simulink model "ecu_mode"  (R2026a)
settings: Solver=FixedStepDiscrete  StopTime=10  FixedStep=0.001  SampleTimeConstraint=STIndependent
Description:
  | Engine state machine. Source of truth for firmware/gen/ecu_mode.
settings Model: Creator=jj1001000  LastModifiedBy=jj1001000
settings OptimizationCC: DefaultUnderspecifiedDataType=single
settings DebuggingCC: ParameterPrecisionLossMsg=none
settings HardwareCC: ProdLargestAtomicInteger=Long  ProdLargestAtomicFloat=Double  ProdHWDeviceType=ARM Compatible->ARM Cortex-M
settings RTWCC: SystemTargetFile=ert.tlc  GenCodeOnly=on  Description=Embedded Coder
settings ERTTargetCC: UtilityFuncGeneration=Shared location  IncludeMdlTerminateFcn=off  CodeInterfacePackaging=Reusable function  SupportNonFinite=off

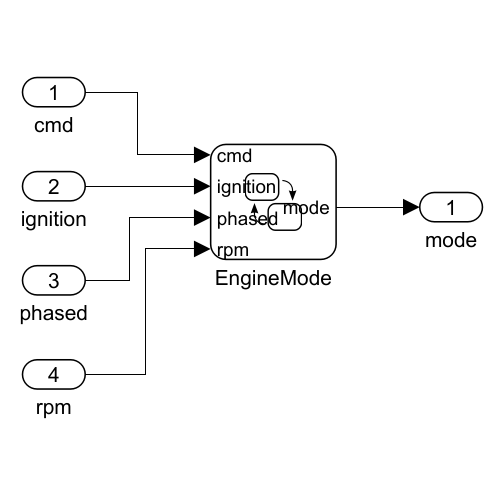
[thumbnail: Simulink's stored preview of the top-level diagram]
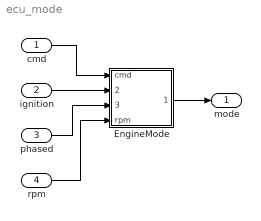
== system ecu_mode ==
  cmd : Inport  OutDataTypeStr=uint8
  ignition : Inport  Port=2  OutDataTypeStr=uint8
  phased : Inport  Port=3  OutDataTypeStr=uint8
  rpm : Inport  Port=4  OutDataTypeStr=single
  EngineMode : Stateflow chart  TreatAsAtomicUnit=on
  mode : Outport  OutDataTypeStr=uint8
  wires:
  cmd/1 -> EngineMode/1(cmd)
  ignition/1 -> EngineMode/2(ignition)
  EngineMode/1(mode) -> mode/1
  rpm/1 -> EngineMode/4(rpm)
  phased/1 -> EngineMode/3(phased)

== stateflow chart ecu_mode/EngineMode ==
  settings: updateMethod=DISCRETE  executeAtInitialization=1
  state Engine
    state OFF
      entry: mode = uint8(0);
    state WAIT
      entry: mode = uint8(1);
    state CRANK
      entry: mode = uint8(2);
    state RUN
      entry: mode = uint8(3);
    Engine -> Engine [order 1] : [cmd == 5]
    (default) -> OFF
    OFF -> WAIT : [cmd == 1 && ignition ~= 0]
    WAIT -> CRANK : [cmd == 2]
    CRANK -> RUN : [cmd == 3 && phased ~= 0 && rpm >= single(400)]
  state SHUTDOWN
    entry: mode = uint8(4); low = uint16(0);
    during:
    if cmd == 1
    if ignition ~= 0
    low = uint16(0);
    elseif rpm == 0
    low = min(low + 1, uint16(500));
    else
    low = uint16(0);
    end
    end
  (default) -> Engine : {low = uint16(0);}
  SHUTDOWN -> Engine [order 1] : [cmd == 5]
  Engine -> SHUTDOWN [order 1] : [cmd == 4]
  SHUTDOWN -> Engine [order 2] : [cmd == 1 && ignition ~= 0 && low >= uint16(500)]
  data: cmd input uint8; ignition input uint8; phased input uint8; rpm input single; mode output uint8; low local uint16
